simulink model "Supervisory"  (R2022b)
settings: Solver=FixedStepDiscrete  StartTime=0.0  StopTime=120  FixedStep=0.001  MaxStep=0.001  RelTol=1e-5
undefined symbols (not defined in the file): reserv_str
libraries: sldvlib x3, simulink x1
settings Model: Creator=szhang  LastModifiedBy=ppatel
settings SolverCC: AlgebraicLoopSolver=TrustRegion
settings DataIOCC: InitialState=simState  LimitDataPoints=on  SaveFinalState=on  SaveOutput=off  SaveTime=off
settings OptimizationCC: DefaultParameterBehavior=Inlined  UseDivisionForNetSlopeComputation=on  UseFloatMulNetSlope=on  InlineInvariantSignals=on  PassReuseOutputArgsAs=Individual arguments  ZeroExternalMemoryAtStartup=off  ZeroInternalMemoryAtStartup=off  NoFixptDivByZeroProtection=on  EfficientFloat2IntCast=on  LifeSpan=Inf  EfficientTunableParamExpr=on
settings DebuggingCC: SignalRangeChecking=error  SolverPrmCheckMsg=warning  IntegerOverflowMsg=error  ParameterTunabilityLossMsg=error  UnconnectedInputMsg=warning  UnconnectedOutputMsg=warning  UnconnectedLineMsg=warning  AssertControl=DisableAll  SFUnexpectedBacktrackingDiag=warning  SFNoUnconditionalDefaultTransitionDiag=warning  SFUnreachableExecutionPathDiag=error  SFExecutionAtInitializationDiag=none  SFMachineParentedDataDiag=warning  ArithmeticOperatorsInVariantConditions=warning
settings HardwareCC: ProdLongLongMode=on
settings ModelReferenceCC: EnableRefExpFcnMdlSchedulingChecks=on  PropagateSignalLabelsOutOfModel=off
settings SFSimCC: SimUseLocalCustomCode=off  MATLABDynamicMemAlloc=off  CustomCodeUndefinedFunction=UseInterfaceOnly
settings RTWCC: Description=Embedded Coder  SystemTargetFile=ert.tlc  TemplateMakefile=ert_default_tmf  GenerateReport=on  RTWUseLocalCustomCode=off  IncludeHyperlinkInReport=on  LaunchReport=on  PortableWordSizes=on  GenerateTraceInfo=on  GenerateTraceReport=on  GenerateTraceReportSl=on  GenerateTraceReportSf=on  GenerateTraceReportEml=on  GenerateCodeMetricsReport=on
settings CodeAppCC: ForceParamTrailComments=on  IgnoreCustomStorageClasses=off  OperatorAnnotations=on  SimulinkDataObjDesc=on  SFDataObjDesc=on  MATLABFcnDesc=on  CustomSymbolStrGlobalVar=rt$N$M  CustomSymbolStrType=$N$M  CustomSymbolStrFcn=$N$M$F  CustomSymbolStrMacro=$N$M  InsertBlockDesc=on  StateflowObjectComments=on  MATLABSourceComments=on  ReqsInCode=on
settings ERTTargetCC: UtilityFuncGeneration=Shared location  MultiwordLength=2048  GenerateSampleERTMain=on  CombineOutputUpdateFcns=off  CombineSignalStateStructs=on  SuppressErrorStatus=on  SupportAbsoluteTime=off  SupportNonFinite=off  SupportComplex=off  ParenthesesLevel=Maximum  CastingMode=Standards  GenerateSharedConstants=off  InlinedParameterPlacement=NonHierarchical  ERTCustomFileTemplate=example_file_process.tlc  ERTFilePackagingFormat=CompactWithDataFile  EnableSignedLeftShifts=off  EnableSignedRightShifts=off
settings ConfigComp: CovEnable=on  CovScope=ReferencedModels  CovIncludeTopModel=off  CovMetricSettings=dcmw  CovHTMLOptions=-sRT=1 -sVT=0 -aTS=1 -bRG=1 -bTC=1 -hTR=0 -nFC=0 -nFD=1 -scm=1 -bcm=1 -xEv=0 -xEM=0  CovSaveCumulativeToWorkspaceVar=on  CovSaveSingleToWorkspaceVar=on  CovCumulativeReport=on  CovModelRefEnable=on  CovExternalEMLEnable=off  CovSFcnEnable=off  DVTestSuiteOptimization=CombinedObjectives (Nonlinear Extended)  DVDesignMinMaxCheck=on  DVHarnessSource=Signal Editor  PSOpenProjectManager=on  PSResultDir=ps_results_$ModelName$  PSAutoStubLUT=on
settings SimscapeCC: SimscapeNormalizeSystem=off  SimscapeLogType=all  SimscapeLogLimitData=off

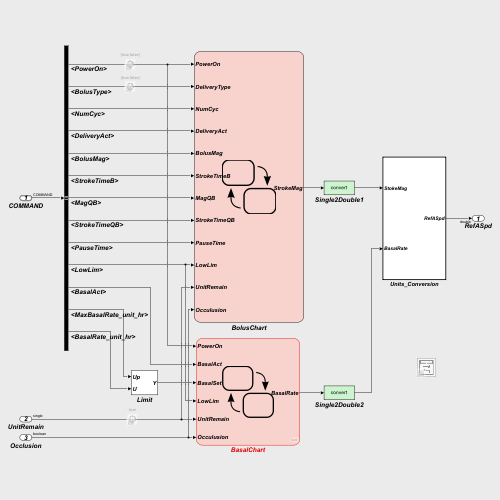
[thumbnail: Simulink's stored preview of the top-level diagram]
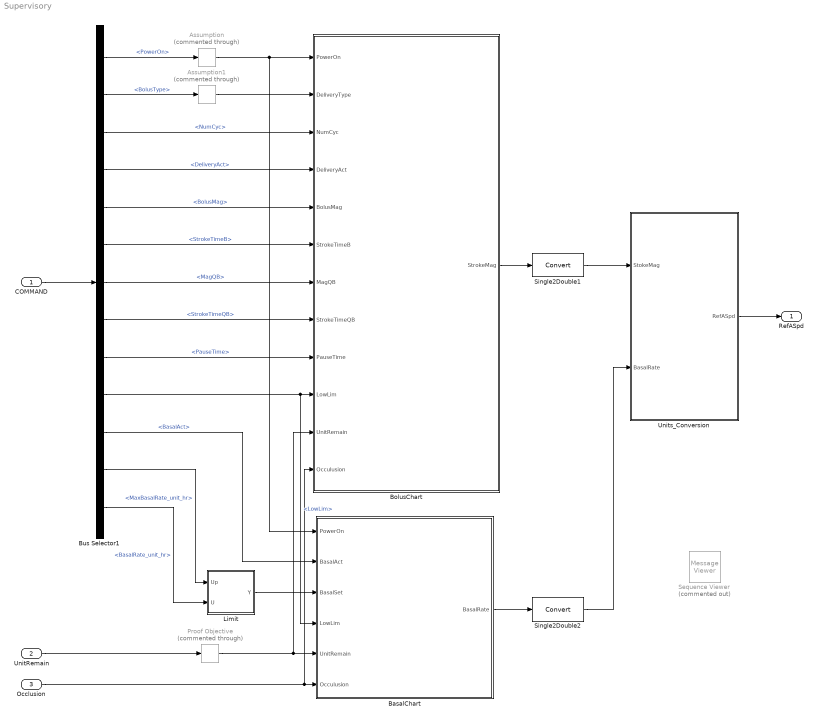
== system Supervisory ==
  COMMAND : Inport  OutDataTypeStr=Bus: COMMAND  PortDimensions=1  BusOutputAsStruct=on
  UnitRemain : Inport  Port=2  OutDataTypeStr=single  PortDimensions=1  SampleTime=0.001
  Occlusion : Inport  Port=3  OutDataTypeStr=boolean  PortDimensions=1  SampleTime=0.001
  Assumption : sldvlib/Objectives and Constraints/Assumption  Commented=through  enabled=on  customAVTBlockType=Assumption  intervals={true,false}  initial=off  dispValues=on  outEnabled=on
      settings: AttributesFormatString=%<intervals>
  Assumption1 : sldvlib/Objectives and Constraints/Assumption  Commented=through  enabled=on  customAVTBlockType=Assumption  intervals={true,false}  initial=off  dispValues=on  outEnabled=on
      settings: AttributesFormatString=%<intervals>
  BasalChart : Stateflow chart  TreatAsAtomicUnit=on
  BolusChart : Stateflow chart  TreatAsAtomicUnit=on  SystemSampleTime=0.001
  Bus Selector1 : BusSelector  OutputSignals=PowerOn,BolusType,NumCyc,DeliveryAct,BolusMag,StrokeTimeB,MagQB,StrokeTimeQB,PauseTime,LowLim,BasalAct,MaxBasalRate_unit_hr,BasalRate_unit_hr
  Limit : Subsystem
  Proof Objective : sldvlib/Objectives and Constraints/Proof Objective  Commented=through  enabled=on  customAVTBlockType=Proof Objective  intervals=true  dispValues=on  outEnabled=on  enableStopSim=off
      settings: AttributesFormatString=%<intervals>
  Sequence Viewer : MessageViewer  Commented=on  History=25000
  Single2Double1 : DataTypeConversion  SaturateOnIntegerOverflow=off  RndMeth=Floor
  Single2Double2 : DataTypeConversion  SaturateOnIntegerOverflow=off  RndMeth=Floor
  Units_Conversion : Subsystem  TreatAsAtomicUnit=on
  RefASpd : Outport  OutMin=-25000  OutMax=25000  OutDataTypeStr=double  PortDimensions=1  SampleTime=0.001  VectorParamsAs1DForOutWhenUnconnected=off
  wires:
  Bus Selector1/3 -> BolusChart/3(NumCyc)  "<NumCyc>"
  Bus Selector1/1 -> Assumption/1  "<PowerOn>"
  Bus Selector1/4 -> BolusChart/4(DeliveryAct)  "<DeliveryAct>"
  Bus Selector1/2 -> Assumption1/1  "<BolusType>"
  Bus Selector1/7 -> BolusChart/7(MagQB)  "<MagQB>"
  Bus Selector1/9 -> BolusChart/9(PauseTime)  "<PauseTime>"
  Bus Selector1/6 -> BolusChart/6(StrokeTimeB)  "<StrokeTimeB>"
  Bus Selector1/8 -> BolusChart/8(StrokeTimeQB)  "<StrokeTimeQB>"
  Occlusion/1 -> BasalChart/6(Occulusion), BolusChart/12(Occulusion)
  Single2Double1/1 -> Units_Conversion/1(StokeMag)
  BasalChart/1(BasalRate) -> Single2Double2/1
  BolusChart/1(StrokeMag) -> Single2Double1/1
  Single2Double2/1 -> Units_Conversion/2(BasalRate)
  UnitRemain/1 -> Proof Objective/1
  Bus Selector1/12 -> Limit/1(Up)  "<MaxBasalRate_unit_hr>"
  Bus Selector1/13 -> Limit/2(U)  "<BasalRate_unit_hr>"
  Limit/1(Y) -> BasalChart/3(BasalSet)
  COMMAND/1 -> Bus Selector1/1
  Bus Selector1/5 -> BolusChart/5(BolusMag)  "<BolusMag>"
  Bus Selector1/10 -> BolusChart/10(LowLim), BasalChart/4(LowLim)  "<LowLim>"
  Bus Selector1/11 -> BasalChart/2(BasalAct)  "<BasalAct>"
  Units_Conversion/1(RefASpd) -> RefASpd/1
  Proof Objective/1 -> BasalChart/5(UnitRemain), BolusChart/11(UnitRemain)
  Assumption/1 -> BolusChart/1(PowerOn), BasalChart/1(PowerOn)
  Assumption1/1 -> BolusChart/2(DeliveryType)

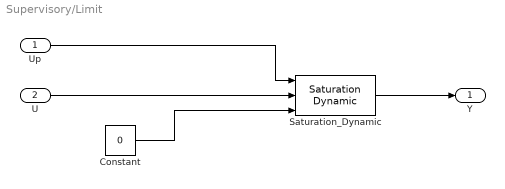
== system Supervisory/Limit ==
  Up : Inport
  U : Inport  Port=2
  Constant : Constant  Value=0  OutDataTypeStr=single
  Saturation_Dynamic : simulink/Discontinuities/Saturation Dynamic  OutMin=0  OutMax=2  OutDataTypeStr=Inherit: Same as second input  OutDataType=fixdt(1, 16)  OutScaling=2^-10  DoSatur=off
  Y : Outport  VectorParamsAs1DForOutWhenUnconnected=off
  wires:
  U/1 -> Saturation_Dynamic/2
  Up/1 -> Saturation_Dynamic/1
  Saturation_Dynamic/1 -> Y/1
  Constant/1 -> Saturation_Dynamic/3

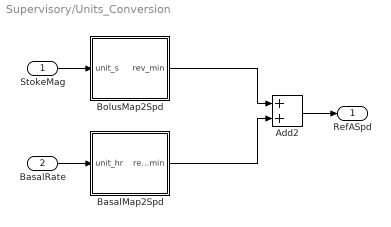
== system Supervisory/Units_Conversion ==
  StokeMag : Inport  OutMin=0  OutMax=15
  BasalRate : Inport  Port=2  OutMin=0  OutMax=2
  Add2 : Sum
  BasalMap2Spd : Subsystem
  BolusMap2Spd : Subsystem
  RefASpd : Outport  OutMin=-25000  OutMax=25000  VectorParamsAs1DForOutWhenUnconnected=off
  wires:
  Add2/1 -> RefASpd/1
  BasalRate/1 -> BasalMap2Spd/1(unit_hr)
  StokeMag/1 -> BolusMap2Spd/1(unit_s)
  BolusMap2Spd/1(rev_min) -> Add2/1
  BasalMap2Spd/1(rev_min) -> Add2/2

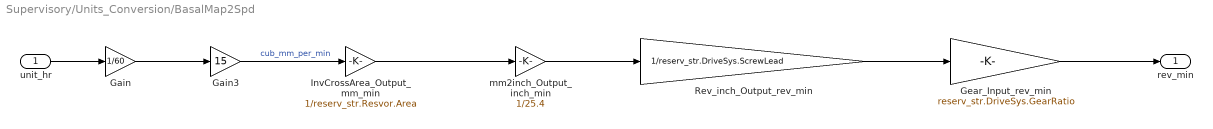
== system Supervisory/Units_Conversion/BasalMap2Spd ==
  unit_hr : Inport
  Gain : Gain  Gain=1/60
  Gain3 : Gain  Gain=15
  Gear_Input_rev_min : Gain  Gain=reserv_str.DriveSys.GearRatio
  InvCrossArea_Output_mm_min : Gain  Gain=1/reserv_str.Resvor.Area
  Rev_inch_Output_rev_min : Gain  Gain=1/reserv_str.DriveSys.ScrewLead
  mm2inch_Output_inch_min : Gain  Gain=1/25.4
  rev_min : Outport  VectorParamsAs1DForOutWhenUnconnected=off
  wires:
  Gear_Input_rev_min/1 -> rev_min/1
  Rev_inch_Output_rev_min/1 -> Gear_Input_rev_min/1
  InvCrossArea_Output_mm_min/1 -> mm2inch_Output_inch_min/1
  unit_hr/1 -> Gain/1
  mm2inch_Output_inch_min/1 -> Rev_inch_Output_rev_min/1
  Gain3/1 -> InvCrossArea_Output_mm_min/1  "cub_mm_per_min"
  Gain/1 -> Gain3/1

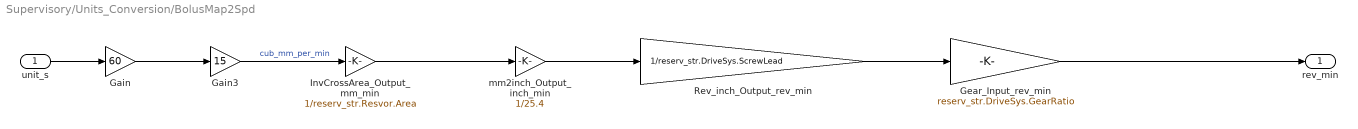
== system Supervisory/Units_Conversion/BolusMap2Spd ==
  unit_s : Inport
  Gain : Gain  Gain=60
  Gain3 : Gain  Gain=15
  Gear_Input_rev_min : Gain  Gain=reserv_str.DriveSys.GearRatio
  InvCrossArea_Output_mm_min : Gain  Gain=1/reserv_str.Resvor.Area
  Rev_inch_Output_rev_min : Gain  Gain=1/reserv_str.DriveSys.ScrewLead
  mm2inch_Output_inch_min : Gain  Gain=1/25.4
  rev_min : Outport  VectorParamsAs1DForOutWhenUnconnected=off
  wires:
  Gear_Input_rev_min/1 -> rev_min/1
  Gain/1 -> Gain3/1
  Gain3/1 -> InvCrossArea_Output_mm_min/1  "cub_mm_per_min"
  mm2inch_Output_inch_min/1 -> Rev_inch_Output_rev_min/1
  unit_s/1 -> Gain/1
  InvCrossArea_Output_mm_min/1 -> mm2inch_Output_inch_min/1
  Rev_inch_Output_rev_min/1 -> Gear_Input_rev_min/1

== stateflow chart Supervisory/BolusChart ==
  state NormalBolusMode
    state OcculusioOccur
    state UnitRemainLow
    state NumCycFinished
    state Deliver
      entry:
      StrokeMag = BolusMag/StrokeTimeB;
    state Active
      entry:
      i = int8(0);
    state Pause
      entry:
      StrokeMag = single(0);
    state Inactive
      entry:
      StrokeMag = single(0);
    OcculusioOccur -> (junction 336)
    (junction 336) -> NormalBolusMode.Inactive
    (junction 342) -> OcculusioOccur [order 2]
    UnitRemainLow -> (junction 337)
    (junction 337) -> NormalBolusMode.Inactive
    (junction 341) -> UnitRemainLow [order 2]
    NumCycFinished -> (junction 338)
    (junction 338) -> NormalBolusMode.Inactive
    (junction 340) -> NumCycFinished [order 2]
    (default) -> NormalBolusMode.Inactive
    Deliver -> (junction 339) : after(StrokeTimeB,sec)
    (junction 339) -> (junction 340) : {i = i + 1;}
    (junction 340) -> (junction 341) [order 1] : [i<NumCyc]
    (junction 341) -> (junction 342) [order 1] : [UnitRemain>=LowLim+BolusMag]
    (junction 342) -> Pause [order 1] : [Occulusion==false]
    NormalBolusMode.Inactive -> (junction 343) : [(UnitRemain>LowLim+BolusMag)&&Occulusion==false]
    (junction 343) -> NormalBolusMode.Active : [DeliveryAct == true]
    NormalBolusMode.Active -> Deliver [order 1] : [i<NumCyc]
    Pause -> Deliver : after(PauseTime,sec)
    NormalBolusMode.Active -> NormalBolusMode.Inactive [order 2] : [UnitRemain<LowLim+BolusMag||Occulusion==true]
  state Off
  state Armed
  state QuickBolusMode
    state Deliver1
      entry:
      StrokeMag = MagQB (1)/StrokeTimeQB(1);
    state Pause1
      entry:
      StrokeMag = single(0);
    state Inactive
      entry:
      StrokeMag = single(0);
    state Active
      entry:
      i = int8(0);
    state Deliver2
      entry:
      StrokeMag = MagQB(2)/StrokeTimeQB(2);
    state Pause2
      entry:
      StrokeMag = single(0);
    state Deliver3
      entry:
      StrokeMag = MagQB(3)/StrokeTimeQB(3);
    state Pause3
      entry:
      StrokeMag = single(0);
    state Deliver4
      entry:
      StrokeMag = MagQB(4)/StrokeTimeQB(4);
    state Pause4
      entry:
      StrokeMag = single(0);
    (junction 284) -> (junction 283)
    (junction 283) -> Deliver1
    Pause4 -> (junction 284) : after(PauseTime,sec)
    (default) -> QuickBolusMode.Inactive
    QuickBolusMode.Inactive -> (junction 285) : [UnitRemain>LowLim+sum(MagQB)]
    (junction 285) -> QuickBolusMode.Active : [DeliveryAct == true]
    QuickBolusMode.Active -> Deliver1
    Deliver1 -> Pause1 : after(StrokeTimeQB(1),sec)
    Pause1 -> Deliver2 : after(PauseTime,sec)
    (junction 295) -> QuickBolusMode.Inactive
    (junction 292) -> QuickBolusMode.Inactive
    (junction 290) -> QuickBolusMode.Inactive
    Deliver2 -> Pause2 : after(StrokeTimeQB(2),sec)
    Pause2 -> Deliver3 : after(PauseTime,sec)
    Deliver3 -> Pause3 : after(StrokeTimeQB(3),sec)
    Pause3 -> Deliver4 : after(PauseTime,sec)
    Deliver4 -> (junction 286) : after(StrokeTimeQB(4),sec)
    (junction 286) -> (junction 287) : {i=i+1;}
    (junction 287) -> (junction 288) [order 1] : [i<NumCyc]
    (junction 288) -> (junction 289) [order 1] : [UnitRemain>=LowLim+sum(MagQB)]
    (junction 289) -> Pause4 [order 1] : [Occulusion==false]
    (junction 287) -> (junction 291) [order 2]
    (junction 288) -> (junction 293) [order 2]
    (junction 289) -> (junction 294) [order 2]
    (junction 291) -> (junction 290)
    (junction 293) -> (junction 292)
    (junction 294) -> (junction 295)
  (default) -> Off
  Off -> Armed : [PowerOn ==true]
  Armed -> Off [order 1] : [PowerOn==false]
  Armed -> NormalBolusMode [order 2] : [DeliveryType ==1]
  NormalBolusMode -> Armed : [DeliveryType~=1]
  Armed -> QuickBolusMode [order 3] : [DeliveryType==2]
  QuickBolusMode -> Armed : [DeliveryType~=2]
  data: PowerOn input boolean size=1 [0..1]; DeliveryType input int8 size=1 [0..2]; NumCyc input int8 size=1 [0..100]; DeliveryAct input boolean size=1 [0..1]; BolusMag input single size=1 [0..3]; StrokeMag output single size=1 [0..15]; i local int8 size=1; StrokeTimeB input single size=1 [0.2..5]; MagQB input single [0..3]; StrokeTimeQB input single [0.2..5]; PauseTime input single size=1 [0..100]; LowLim input single size=1 [0..100]; UnitRemain input single size=1 [0..201]; Occulusion input boolean size=1 [0..1]

== stateflow chart Supervisory/BasalChart ==
  state Off
  state On
  state BasalOff
    during:
    BasalRate = single(0);
  state BasalOn
    during:
    BasalRate = BasalSet;
    exit:
    BasalRate = single(0);
  (default) -> Off
  Off -> On : [PowerOn ==true]
  On -> Off [order 1] : [PowerOn==false]
  On -> BasalOff [order 2] : [(UnitRemain>LowLim)&&Occulusion==false]
  BasalOff -> BasalOn [order 2] : [BasalAct==true]
  BasalOn -> BasalOff [order 3] : [PowerOn==false]
  BasalOff -> On [order 3] : [PowerOn==false]
  BasalOn -> BasalOff [order 1] : [BasalAct==false]
  BasalOn -> BasalOff [order 2] : [UnitRemain<LowLim||Occulusion==true]
  BasalOff -> On [order 1] : [UnitRemain<LowLim||Occulusion==true]
  data: PowerOn input boolean [0..1]; BasalAct input boolean [0..1]; BasalSet input single [0..2]; LowLim input single [0..100]; UnitRemain input single [0..201]; BasalRate output single [0..2]; Occulusion input boolean [0..1]
